simulink model "total_acceleration_test_drvr"  (Simulink 4.00)
settings: Solver=ode45  StartTime=0.0  StopTime=3  RelTol=1e-3
undefined symbols (not defined in the file or in its folder): getElem, plumbbobg, rpy2dcm, skew
libraries: simulink3 x1
settings Model: Creator=mcar  LastModifiedBy=mcar  BlockReductionOpt=off

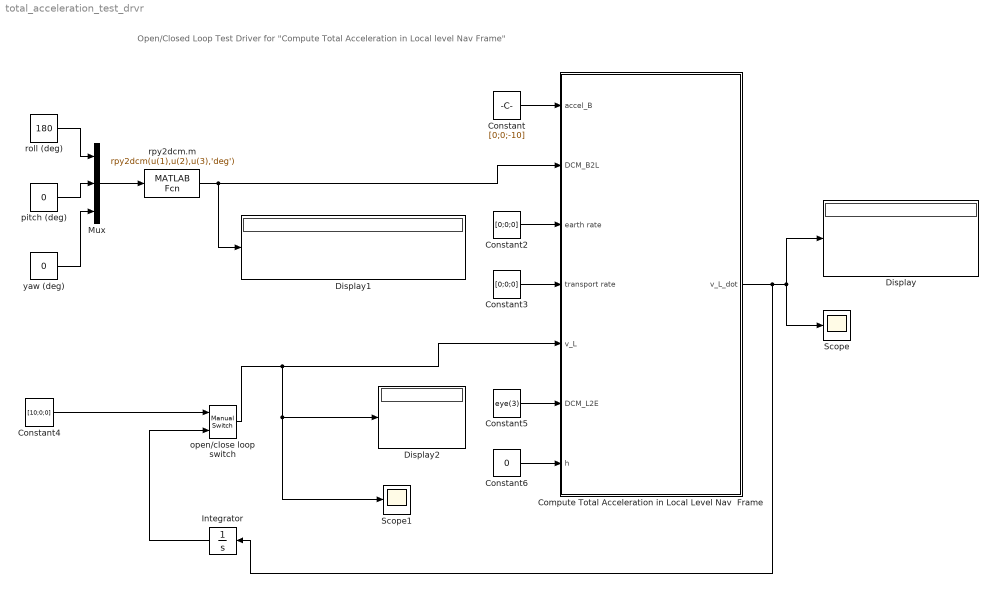
== system total_acceleration_test_drvr ==
  note: Open/Closed Loop Test Driver
      | for "Compute Total Acceleration
      | in Local level Nav Frame"
  Compute Total Acceleration in Local Level Nav  Frame : Subsystem
      settings: RTWFcnNameOpts=Auto  RTWFileNameOpts=Auto
  Constant : Constant  Value=[0;0;-10]  VectorParams1D=off
  Constant2 : Constant  Value=[0;0;0]  VectorParams1D=off
  Constant3 : Constant  Value=[0;0;0]  VectorParams1D=off
  Constant4 : Constant  Value=[10;0;0]  VectorParams1D=off
  Constant5 : Constant  Value=eye(3)  VectorParams1D=off
  Constant6 : Constant  Value=0  VectorParams1D=off
  Display : Display
  Display1 : Display
      settings: Format=short
  Display2 : Display
      settings: Format=short
  Integrator : Integrator  Orientation=left  ExternalReset=none  InitialConditionSource=internal  InitialCondition=0  LimitOutput=off  UpperSaturationLimit=inf  LowerSaturationLimit=-inf  ShowSaturationPort=off  ShowStatePort=off  AbsoluteTolerance=auto
  Mux : Mux  Inputs=3
  Scope : Scope
      settings: TimeRange=auto  YMin=-5  YMax=5  SaveToWorkspace=off  SaveName=ScopeData  LimitDataPoints=on  MaxDataPoints=5000
  Scope1 : Scope
      settings: TimeRange=auto  YMin=-5  YMax=5  SaveToWorkspace=off  LimitDataPoints=on  MaxDataPoints=5000
  open/close loop switch : simulink3/Nonlinear/Manual Switch  sw=0  action=0
  pitch (deg) : Constant  Value=0  VectorParams1D=off
  roll (deg) : Constant  Value=180  VectorParams1D=off
  rpy2dcm.m : MATLABFcn  MATLABFcn=rpy2dcm(u(1),u(2),u(3),'deg')  OutputDimensions=-1  OutputSignalType=auto  Output1D=off
  yaw (deg) : Constant  Value=0  VectorParams1D=off
  wires:
  Constant6/1 -> Compute Total Acceleration in Local Level Nav  Frame/7(h)
  Constant5/1 -> Compute Total Acceleration in Local Level Nav  Frame/6(DCM_L2E)
  Constant3/1 -> Compute Total Acceleration in Local Level Nav  Frame/4(transport rate)
  Constant2/1 -> Compute Total Acceleration in Local Level Nav  Frame/3(earth rate)
  rpy2dcm.m/1 -> Compute Total Acceleration in Local Level Nav  Frame/2(DCM_B2L), Display1/1
  Constant/1 -> Compute Total Acceleration in Local Level Nav  Frame/1(accel_B)
  Compute Total Acceleration in Local Level Nav  Frame/1(v_L_dot) -> Display/1, Scope/1, Integrator/1
  roll (deg)/1 -> Mux/1
  Mux/1 -> rpy2dcm.m/1
  pitch (deg)/1 -> Mux/2
  yaw (deg)/1 -> Mux/3
  Constant4/1 -> open/close loop switch/1
  Integrator/1 -> open/close loop switch/2
  open/close loop switch/1 -> Compute Total Acceleration in Local Level Nav  Frame/5(v_L), Display2/1, Scope1/1

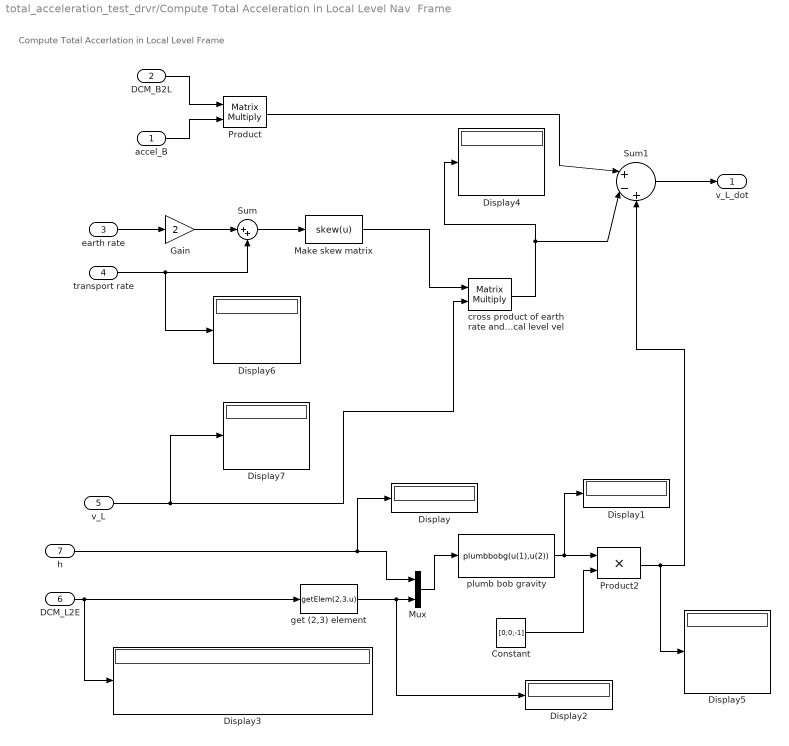
== system total_acceleration_test_drvr/Compute Total Acceleration in Local Level Nav  Frame ==
  note: Compute Total Accerlation in
      | Local Level Frame
  accel_B : Inport  Port=1
  DCM_B2L : Inport  Port=2
  earth rate : Inport  Port=3
  transport rate : Inport  Port=4
  v_L : Inport  Port=5
  DCM_L2E : Inport  Port=6
  h : Inport  Port=7
  Constant : Constant  Value=[0;0;-1]  VectorParams1D=off
  Display{,1..7} (8 alike) : Display
      settings: Format=short
  Gain : Gain  Gain=2  Multiplication=Element-wise(K.*u)  SaturateOnIntegerOverflow=on
  Make skew matrix : MATLABFcn  MATLABFcn=skew(u)  OutputDimensions=-1  OutputSignalType=auto  Output1D=off
  Mux : Mux  Inputs=2
  Product : Product  Inputs=2  Multiplication=Matrix(*)  SaturateOnIntegerOverflow=on
  Product2 : Product  Inputs=2  Multiplication=Element-wise(.*)  SaturateOnIntegerOverflow=on
  Sum : Sum  Inputs=|++  SaturateOnIntegerOverflow=on
  Sum1 : Sum  Inputs=|+-+  SaturateOnIntegerOverflow=on
  cross product of earth rate and  transport rates  with local level vel : Product  Inputs=2  Multiplication=Matrix(*)  SaturateOnIntegerOverflow=on
  get (2,3) element : MATLABFcn  MATLABFcn=getElem(2,3,u)  OutputDimensions=-1  OutputSignalType=auto  Output1D=off
  plumb bob gravity : MATLABFcn  MATLABFcn=plumbbobg(u(1),u(2))  OutputDimensions=-1  OutputSignalType=auto  Output1D=on
  v_L_dot : Outport  Port=1
  wires:
  Sum1/1 -> v_L_dot/1
  Product/1 -> Sum1/1
  cross product of earth rate and  transport rates  with local level vel/1 -> Sum1/2, Display4/1
  v_L/1 -> cross product of earth rate and  transport rates  with local level vel/2, Display7/1
  Make skew matrix/1 -> cross product of earth rate and  transport rates  with local level vel/1
  Sum/1 -> Make skew matrix/1
  transport rate/1 -> Sum/2, Display6/1
  Gain/1 -> Sum/1
  earth rate/1 -> Gain/1
  accel_B/1 -> Product/2
  DCM_B2L/1 -> Product/1
  DCM_L2E/1 -> get (2,3) element/1, Display3/1
  h/1 -> Mux/1, Display/1
  get (2,3) element/1 -> Mux/2, Display2/1
  Mux/1 -> plumb bob gravity/1
  Constant/1 -> Product2/2
  plumb bob gravity/1 -> Product2/1, Display1/1
  Product2/1 -> Sum1/3, Display5/1
